simulink model "chapter4_cascaded_nonlinear_closed_pid"  (R2023b)
settings: Solver=ode45  StartTime=0.0  StopTime=100  FixedStep=0.001  MaxStep=1e-3  RelTol=1e-3  EnableMultiTasking=on
values from neighbouring files (symbols this model uses):
  B = 735.75    [rovmodel75kg.mat]
  DL = [3.221 0 0 0 0 0 0 3.291 0 0 0 0 ... (36 elements, 6x6)]    [rovmodel75kg.mat]
  DQ = [105.3 0 0 0 0 0 0 139.6 0 0 0 0 ... (36 elements, 6x6)]    [rovmodel75kg.mat]
  I = [2.51  0  0; 0  3.38  0.01; 0  0.01  1.73]    [rovmodel75kg.mat]
  m = [75  0  0; 0  75  0; 0  0  75]    [rovmodel75kg.mat]
  M = [75 0 0 0 0 0 0 75 0 0 0 0 ... (36 elements, 6x6)]    [rovmodel75kg.mat]
  Ma = [-20.392 0 0 0 0 0 0 -53.435 0 0 0 0 ... (36 elements, 6x6)]    [rovmodel75kg.mat]
  rg = [0 0 0]    [rovmodel75kg.mat]
  W = 735.75    [rovmodel75kg.mat]
  zb = -0.397    [rovmodel75kg.mat]
  zg = 0    [rovmodel75kg.mat]
libraries: simulink_need_slupdate x12
settings Model: Creator=Joshua cheng  LastModifiedBy=yhm
settings SolverCC: AlgebraicLoopSolver=TrustRegion
settings DataIOCC: LimitDataPoints=on  SaveFormat=Array  SignalLoggingSaveFormat=ModelDataLogs  ReturnWorkspaceOutputs=off
settings OptimizationCC: BlockReduction=off  OptimizeBlockIOStorage=off  BufferReuse=off  GlobalBufferReuse=off  ExpressionFolding=off  ExpressionDepthLimit=2147483647  LocalBlockOutputs=off  LifeSpan=inf  OptimizeDataStoreBuffers=off  BusAssignmentInplaceUpdate=off
settings DebuggingCC: SaveWithParameterizedLinksMsg=none  UnderspecifiedInitializationDetection=Classic  MergeDetectMultiDrivingBlocksExec=none  SolverPrmCheckMsg=warning  FcnCallInpInsideContextMsg=warning  UnconnectedInputMsg=warning  UnconnectedOutputMsg=warning  UnconnectedLineMsg=warning  StateNameClashWarn=warning  SFUnexpectedBacktrackingDiag=warning  SFNoUnconditionalDefaultTransitionDiag=warning  SFExecutionAtInitializationDiag=none  ArithmeticOperatorsInVariantConditions=warning
settings HardwareCC: ProdBitPerPointer=32  ProdBitPerSizeT=32  ProdBitPerPtrDiffT=32  ProdLargestAtomicFloat=None  ProdEndianess=BigEndian  ProdWordSize=32  ProdHWDeviceType=Specified  TargetIntDivRoundTo=Zero  TargetEndianess=BigEndian
settings ModelReferenceCC: EnableRefExpFcnMdlSchedulingChecks=on  PropagateSignalLabelsOutOfModel=off
settings SFSimCC: SimUseLocalCustomCode=off  CustomCodeUndefinedFunction=UseInterfaceOnly
settings RTWCC: Description=dSPACE DS1104 Hardware Platform  SystemTargetFile=rti1104.tlc  MakeCommand=make_rti  TemplateMakefile=rti1104.tmf  RTWUseLocalCustomCode=off
settings CodeAppCC: StateflowObjectComments=on
settings STFCustomTargetCC: TargetLangStandard=C89/C90 (ANSI)  MatFileLogging=on  CPPClassGenCompliant=on  GRTInterface=on  SystemTargetFile=rti1104.tlc
settings GRTTargetCC: TargetLangStandard=C89/C90 (ANSI)  ParMdlRefBuildCompliant=off  CompOptLevelCompliant=off  ConcurrentExecutionCompliant=off  CombineOutputUpdateFcns=off  GRTInterface=on  UseToolchainInfoCompliant=off  ExtModeMexFile=noextcomm
settings ConfigComp: CovMetricSettings=dw  CovSaveCumulativeToWorkspaceVar=on  CovSaveSingleToWorkspaceVar=on  CovExternalEMLEnable=off

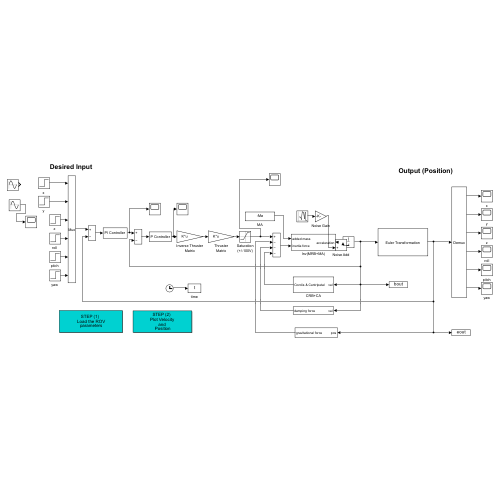
[thumbnail: Simulink's stored preview of the top-level diagram]
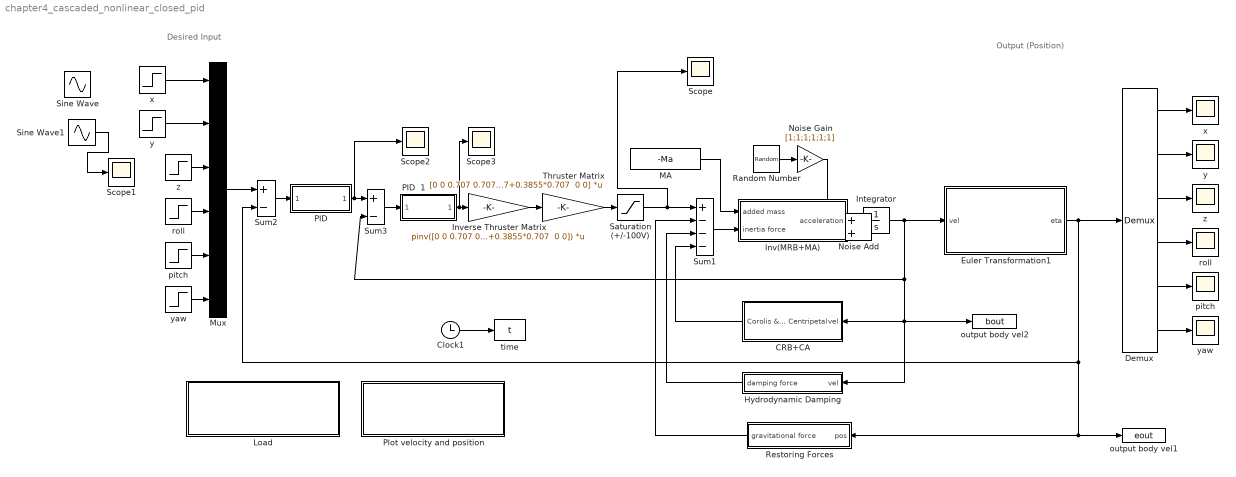
== system chapter4_cascaded_nonlinear_closed_pid ==
  note: Desired Input
  note: Output (Position)
  " Load  " : Subsystem
      settings: OpenFcn=|
      | clc
      | clear all
      | close all
      | load('rovmodel75kg.mat')
      mask Display: disp('STEP (1) \n Load the ROV\n parameters')
  " PID  " : Subsystem  AncestorBlock=|
      | rov_design_analysis/ROV Controller
      | Design
      | Applications/8. PID x 4
      mask Display: disp('PI Controller')
  " PID  1" : Subsystem  AncestorBlock=|
      | rov_design_analysis/ROV Controller
      | Design
      | Applications/8. PID x 4
      mask Display: disp('P Controller')
  CRB+CA : Subsystem
  Clock1 : Clock
  Demux : Demux  Outputs=6
      settings: DisplayOption=none
  Euler Transformation1 : Subsystem  AncestorBlock=rov_design_analysis/Scope Utilities/Euler Transformation
      mask Display: disp('Euler Transformation')
  Hydrodynamic Damping : Subsystem
  Integrator : Integrator  InitialCondition=0.1
  Inv(MRB+MA) : Subsystem
  "Inverse Thruster Matrix " : Gain  Gain=|  Multiplication=Matrix(K*u)  SaturateOnIntegerOverflow=on  OutDataTypeStr=Inherit: Same as input  ParamDataTypeStr=Inherit: Same as input
      | pinv([0 0 0.707 0.707 0 0; 
      |     -0.707 0.707 0.707 -0.707 0 0; 
      |     0.707  0.707  0 0 1 1;
      |     -0.275*0.707+0.4305*0.707 0.275*0.707-0.4305*0.707  0  0  -0.275 0.275;
      |     0.3945*0.707 0.3945*0.707  0.4305*0.707  0.4305*0.707  -0.0355  -0.0355;
      |       -0.3945*0.707  0.3945*0.707  -0.275*0.707-0.3855*0.707  0.275*0.707+0.3855*0.707  0 0])
  MA : Constant  Value=-Ma
  Mux : Mux  Inputs=6
  Noise Add : Sum
  Noise Gain : Gain  Gain=[1;1;1;1;1;1]
  Plot velocity and position : Subsystem  AncestorBlock=|
      | rov_design_analysis/ROV Controller
      | Design
      | Applications/Plot velocity and position
      settings: OpenFcn=|
      | clc
      | 
      | run nonlin_resp6
      mask Display: disp('STEP (2) \n Plot Velocity \n and \n Position')
  Random Number : RandomNumber  Variance=0.001  SampleTime=0.1
  Restoring Forces : Subsystem
  Saturation (+/-100V) : Saturate  UpperLimit=100  LowerLimit=-100
  Scope{,1..3} (4 alike) : Scope
  Sine Wave : Sin  Amplitude=2  Frequency=0.2  Phase=pi/2  SampleTime=0
  Sine Wave1 : Sin  Amplitude=2  Frequency=0.2  SampleTime=0
  Sum1 : Sum  Inputs=+---  InputSameDT=on  SaturateOnIntegerOverflow=on  OutDataTypeStr=Inherit: Same as first input
  Sum2 : Sum  Inputs=+-  InputSameDT=on  SaturateOnIntegerOverflow=on  OutDataTypeStr=Inherit: Same as first input
  Sum3 : Sum  Inputs=+-  InputSameDT=on  SaturateOnIntegerOverflow=on  OutDataTypeStr=Inherit: Same as first input
  "Thruster Matrix " : Gain  Gain=|  Multiplication=Matrix(K*u)  SaturateOnIntegerOverflow=on  OutDataTypeStr=Inherit: Same as input  ParamDataTypeStr=Inherit: Same as input
      | [0 0 0.707 0.707 0 0; 
      |     -0.707 0.707 0.707 -0.707 0 0; 
      |     0.707  0.707  0 0 1 1;
      |     -0.275*0.707+0.4305*0.707 0.275*0.707-0.4305*0.707  0  0  -0.275 0.275;
      |     0.3945*0.707 0.3945*0.707  0.4305*0.707  0.4305*0.707  -0.0355  -0.0355;
      |       -0.3945*0.707  0.3945*0.707  -0.275*0.707-0.3855*0.707  0.275*0.707+0.3855*0.707  0 0]
  output body vel1 : ToWorkspace  VariableName=eout  SampleTime=-1
  output body vel2 : ToWorkspace  VariableName=bout  SampleTime=-1
  pitch : Scope
  "pitch " : Step  Time=0  After=0  SampleTime=0
  roll : Scope
  "roll " : Step  Time=0  After=0  SampleTime=0
  time : ToWorkspace  VariableName=t  SampleTime=-1
  x : Scope
  "x " : Step  Time=0  After=2  SampleTime=0
  y : Scope
  "y " : Step  Time=0  After=2  SampleTime=0
  yaw : Scope
  "yaw " : Step  Time=0  After=0  SampleTime=0
  z : Scope
  "z " : Step  Time=0  After=2  SampleTime=0
  wires:
  Clock1/1 -> time/1
  Euler Transformation1/1("eta ") -> Restoring Forces/1(pos), output body vel1/1, Sum2/2, Demux/1
  MA/1 -> Inv(MRB+MA)/1(added mass)
  CRB+CA/1(Corolis & Centripetal) -> Sum1/4
  Hydrodynamic Damping/1(damping force) -> Sum1/3
  Restoring Forces/1(gravitational force) -> Sum1/2
  Integrator/1 -> CRB+CA/1(vel), Hydrodynamic Damping/1(vel), output body vel2/1, Sum3/2, Euler Transformation1/1(vel)
  Sum1/1 -> Inv(MRB+MA)/2(inertia force)
  "Inverse Thruster Matrix "/1 -> "Thruster Matrix "/1
  "Thruster Matrix "/1 -> Saturation (+/-100V)/1
  "z "/1 -> Mux/3
  "roll "/1 -> Mux/4
  "pitch "/1 -> Mux/5
  "yaw "/1 -> Mux/6
  Demux/6 -> yaw/1
  Demux/3 -> z/1
  Demux/4 -> roll/1
  Demux/5 -> pitch/1
  Demux/2 -> y/1
  Demux/1 -> x/1
  Mux/1 -> Sum2/1
  Sum2/1 -> " PID  "/1(error signal)
  Saturation (+/-100V)/1 -> Scope/1, Sum1/1
  " PID  "/1(control signal) -> Scope2/1, Sum3/1
  " PID  1"/1(control signal) -> Scope3/1, "Inverse Thruster Matrix "/1
  Sum3/1 -> " PID  1"/1(error signal)
  Sine Wave1/1 -> Scope1/1
  "x "/1 -> Mux/1
  "y "/1 -> Mux/2
  Inv(MRB+MA)/1(acceleration) -> Noise Add/1
  Random Number/1 -> Noise Gain/1
  Noise Gain/1 -> Noise Add/2
  Noise Add/1 -> Integrator/1

== system chapter4_cascaded_nonlinear_closed_pid/ Load   ==

== system chapter4_cascaded_nonlinear_closed_pid/ PID   ==
  error signal : Inport
  Demux1 : Demux  Outputs=6
      settings: DisplayOption=none
  Mux2 : Mux  Inputs=6
  PID Controller1 : simulink_need_slupdate/PID Controller  P=2  I=0.5  D=6
  PID Controller2 : simulink_need_slupdate/PID Controller  P=2  I=0.5  D=6
  PID Controller3 : simulink_need_slupdate/PID Controller  P=3  I=0.5  D=6
  PID Controller4 : simulink_need_slupdate/PID Controller  P=3  I=0.5  D=3
  PID Controller5 : simulink_need_slupdate/PID Controller  P=3  I=0.5  D=3
  PID Controller6 : simulink_need_slupdate/PID Controller  P=2  I=0.5  D=6
  control signal : Outport
  wires:
  Mux2/1 -> control signal/1
  error signal/1 -> Demux1/1
  PID Controller2/1 -> Mux2/2
  PID Controller1/1 -> Mux2/1
  Demux1/2 -> PID Controller2/1
  Demux1/1 -> PID Controller1/1
  Demux1/3 -> PID Controller3/1
  PID Controller3/1 -> Mux2/3
  Demux1/6 -> PID Controller6/1
  PID Controller6/1 -> Mux2/6
  Demux1/4 -> PID Controller4/1
  Demux1/5 -> PID Controller5/1
  PID Controller4/1 -> Mux2/4
  PID Controller5/1 -> Mux2/5

== system chapter4_cascaded_nonlinear_closed_pid/ PID  1 ==
  error signal : Inport
  Demux1 : Demux  Outputs=6
      settings: DisplayOption=none
  Mux2 : Mux  Inputs=6
  PID Controller1 : simulink_need_slupdate/PID Controller  P=5  I=0  D=0
  PID Controller2 : simulink_need_slupdate/PID Controller  P=11  I=0  D=0
  PID Controller3 : simulink_need_slupdate/PID Controller  P=12  I=0  D=0
  PID Controller4 : simulink_need_slupdate/PID Controller  P=12  I=0  D=0
  PID Controller5 : simulink_need_slupdate/PID Controller  P=12  I=0  D=0
  PID Controller6 : simulink_need_slupdate/PID Controller  P=11  I=0  D=0
  control signal : Outport
  wires:
  Mux2/1 -> control signal/1
  error signal/1 -> Demux1/1
  PID Controller2/1 -> Mux2/2
  PID Controller1/1 -> Mux2/1
  Demux1/2 -> PID Controller2/1
  Demux1/1 -> PID Controller1/1
  Demux1/3 -> PID Controller3/1
  PID Controller3/1 -> Mux2/3
  Demux1/6 -> PID Controller6/1
  PID Controller6/1 -> Mux2/6
  Demux1/4 -> PID Controller4/1
  Demux1/5 -> PID Controller5/1
  PID Controller4/1 -> Mux2/4
  PID Controller5/1 -> Mux2/5

== system chapter4_cascaded_nonlinear_closed_pid/CRB+CA ==
  vel : Inport
  Add : Sum
  Centripetal & Coriolis : Subsystem  AncestorBlock=rov_design_analysis/ROV Models/1. Six DOF RRC ROV II/Centripetal & Coriolis
      mask Display: disp('CRB')
  Centripetal & Coriolis1 : Subsystem  AncestorBlock=rov_design_analysis/ROV Models/1. Six DOF RRC ROV II/Centripetal & Coriolis
      mask Display: disp('CA')
  Corolis & Centripetal : Outport
  wires:
  vel/1 -> Centripetal & Coriolis/1(vel), Centripetal & Coriolis1/1(vel)
  Add/1 -> Corolis & Centripetal/1
  Centripetal & Coriolis/1(force) -> Add/1
  Centripetal & Coriolis1/1(force) -> Add/2

== system chapter4_cascaded_nonlinear_closed_pid/Euler Transformation1 ==
  vel : Inport
  1/s : Subsystem
  Demux : Demux  Outputs=2
      settings: DisplayOption=none
  Demux1 : Demux  Outputs=2
      settings: DisplayOption=none
  Mux1 : Mux  Inputs=2
  Saturation : Saturate  UpperLimit=360  LowerLimit=-360
  Terminator : Terminator
  Transformation matrix R : Subsystem
      mask Display: disp('Transformation R')
  Transformation matrix T : Subsystem
      mask Display: disp('Transformation T')
  "eta " : Outport  InitialOutput=0
  wires:
  Mux1/1 -> 1/s/1(In1)
  Demux/2 -> Transformation matrix R/1(angular body velocity)
  Demux/1 -> Transformation matrix T/1(translational body velocity)
  vel/1 -> Demux/1
  Demux1/2 -> Transformation matrix T/2(angular position), Transformation matrix R/2(angular position)
  Transformation matrix R/1(angular earth velocity) -> Mux1/2
  Transformation matrix T/1(translational earth velocity) -> Mux1/1
  Demux1/1 -> Terminator/1
  1/s/1(Out1) -> Saturation/1
  Saturation/1 -> Demux1/1, "eta "/1

== system chapter4_cascaded_nonlinear_closed_pid/Hydrodynamic Damping ==
  vel : Inport
  Abs : Abs  SaturateOnIntegerOverflow=off
  Add : Sum
  Constant : Constant  Value=0
  D linear : Gain  Gain=diag(DL)  SaturateOnIntegerOverflow=on  OutDataTypeStr=Inherit: Same as input  ParamDataTypeStr=Inherit: Same as input
  D quadratic : Gain  Gain=diag(DQ)  SaturateOnIntegerOverflow=on  OutDataTypeStr=Inherit: Same as input  ParamDataTypeStr=Inherit: Same as input
  Manual Switch : ManualSwitch  CurrentSetting=0
  Manual Switch1 : ManualSwitch  CurrentSetting=0
  Product : Product  RndMeth=Zero
  damping force : Outport  InitialOutput=0
  wires:
  vel/1 -> D linear/1, Abs/1, Product/2
  D linear/1 -> Manual Switch/1
  Add/1 -> damping force/1
  Abs/1 -> D quadratic/1
  D quadratic/1 -> Product/1
  Manual Switch/1 -> Add/1
  Product/1 -> Manual Switch/2, Manual Switch1/2
  Manual Switch1/1 -> Add/2
  Constant/1 -> Manual Switch1/1

== system chapter4_cascaded_nonlinear_closed_pid/Inv(MRB+MA) ==
  added mass : Inport
  inertia force : Inport  Port=2
  Display : Display
      settings: Decimation=2
  Display2 : Display
      settings: Decimation=2
  Divide : Product  Inputs=/  Multiplication=Matrix(*)
  MRB - open : Constant  Value=M
  Product : Product  Multiplication=Matrix(*)  RndMeth=Zero
  Sum1 : Sum  InputSameDT=on  SaturateOnIntegerOverflow=on  OutDataTypeStr=Inherit: Same as first input
  acceleration : Outport
  wires:
  Divide/1 -> Display/1, Product/1
  Product/1 -> acceleration/1, Display2/1
  inertia force/1 -> Product/2
  added mass/1 -> Sum1/2
  Sum1/1 -> Divide/1
  MRB - open/1 -> Sum1/1

== system chapter4_cascaded_nonlinear_closed_pid/Plot velocity and position ==

== system chapter4_cascaded_nonlinear_closed_pid/Restoring Forces ==
  pos : Inport
  (zg.W - zb.B)cY.sX : Fcn  Expr=((zg * W - zb * B) * cos(u[2])) * sin(u[1])
  (zg.W - zb.B)sY : Fcn  Expr=(zg*W - zb*B)*sin(u[2])
  -(xg.W-xb.B)cY.sX : Fcn  Expr=0
  -cY.cX : Fcn  Expr=0
  -cY.sX : Fcn  Expr=0
  Demux : Demux  Outputs=2
      settings: DisplayOption=none
  Mux1 : Mux  Inputs=6
  Terminator : Terminator
  sY : Fcn  Expr=0
  gravitational force : Outport  InitialOutput=0
  wires:
  Mux1/1 -> gravitational force/1
  Demux/2 -> (zg.W - zb.B)cY.sX/1, (zg.W - zb.B)sY/1, -(xg.W-xb.B)cY.sX/1, sY/1, -cY.sX/1, -cY.cX/1  "pos_2"
  Demux/1 -> Terminator/1  "pos_1"
  pos/1 -> Demux/1
  sY/1 -> Mux1/1
  -cY.sX/1 -> Mux1/2
  -cY.cX/1 -> Mux1/3
  (zg.W - zb.B)cY.sX/1 -> Mux1/4
  (zg.W - zb.B)sY/1 -> Mux1/5
  -(xg.W-xb.B)cY.sX/1 -> Mux1/6

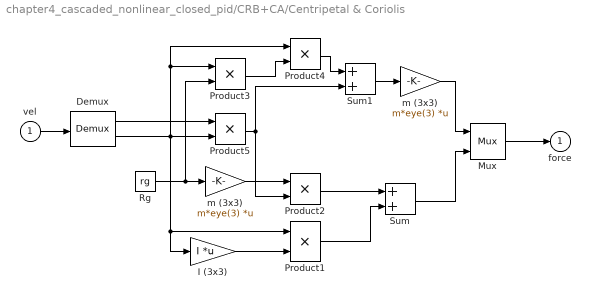
== system chapter4_cascaded_nonlinear_closed_pid/CRB+CA/Centripetal & Coriolis ==
  vel : Inport
  Demux : Demux  Outputs=2
      settings: DisplayOption=none
  "I (3x3) " : Gain  Gain=I  Multiplication=Matrix(K*u)  SaturateOnIntegerOverflow=on  OutDataTypeStr=Inherit: Same as input  ParamDataTypeStr=Inherit: Same as input
  Mux : Mux  Inputs=2
  Product{1..5} (5 alike) : Product  InputSameDT=on  RndMeth=Zero  SaturateOnIntegerOverflow=on  OutDataTypeStr=Inherit: Same as first input
  Rg : Constant  Value=rg
  Sum : Sum  InputSameDT=on  SaturateOnIntegerOverflow=on  OutDataTypeStr=Inherit: Same as first input
  Sum1 : Sum  InputSameDT=on  SaturateOnIntegerOverflow=on  OutDataTypeStr=Inherit: Same as first input
  m (3x3) : Gain  Gain=m*eye(3)  Multiplication=Matrix(K*u)  SaturateOnIntegerOverflow=on  OutDataTypeStr=Inherit: Same as input  ParamDataTypeStr=Inherit: Same as input
  "m (3x3) " : Gain  Gain=m*eye(3)  Multiplication=Matrix(K*u)  SaturateOnIntegerOverflow=on  OutDataTypeStr=Inherit: Same as input  ParamDataTypeStr=Inherit: Same as input
  force : Outport  InitialOutput=0
  wires:
  Product1/1 -> Sum/2
  "m (3x3) "/1 -> Product2/1
  Product2/1 -> Sum/1
  Product3/1 -> Product4/2
  Product4/1 -> Sum1/1
  Product5/1 -> Product2/2, Sum1/2
  Sum1/1 -> m (3x3)/1
  vel/1 -> Demux/1
  m (3x3)/1 -> Mux/1
  Sum/1 -> Mux/2
  Mux/1 -> force/1
  Demux/1 -> Product5/1
  Demux/2 -> Product5/2, Product3/1, Product4/1, Product1/1, "I (3x3) "/1
  Rg/1 -> "m (3x3) "/1, Product3/2
  "I (3x3) "/1 -> Product1/2

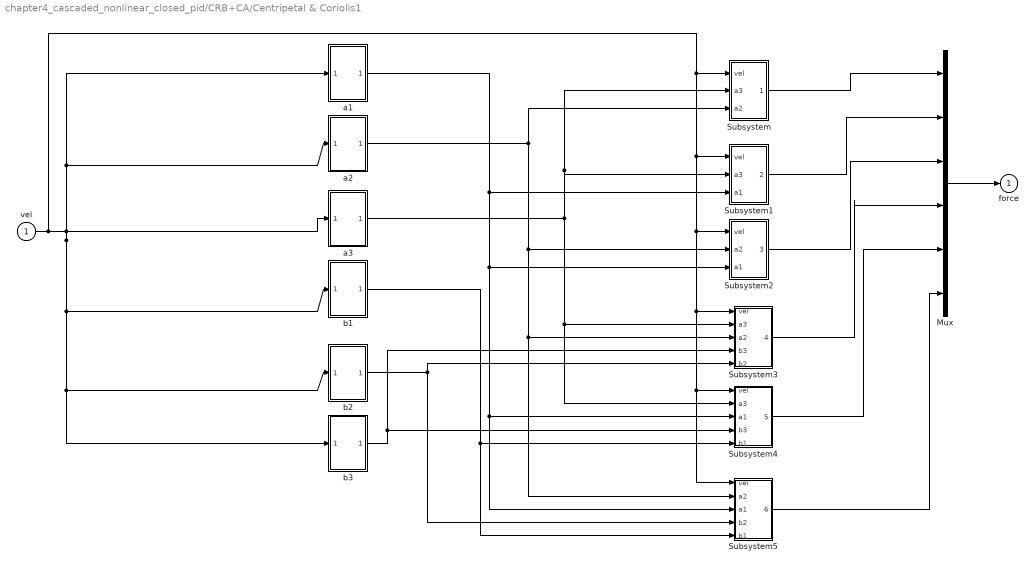
== system chapter4_cascaded_nonlinear_closed_pid/CRB+CA/Centripetal & Coriolis1 ==
  vel : Inport
  Mux : Mux  Inputs=6
  Subsystem : Subsystem
  Subsystem1 : Subsystem
  Subsystem2 : Subsystem
  Subsystem3 : Subsystem
  Subsystem4 : Subsystem
  Subsystem5 : Subsystem
  a1 : Subsystem
      mask Display: disp('Row 1')
  a2 : Subsystem
      mask Display: disp('Row 2')
  a3 : Subsystem
      mask Display: disp('Row 1')
  b1 : Subsystem
      mask Display: disp('Row 2')
  b2 : Subsystem
      mask Display: disp('Row 1')
  b3 : Subsystem
      mask Display: disp('Row 2')
  force : Outport  InitialOutput=0
  wires:
  vel/1 -> a1/1(In1), a2/1(In1), a3/1(In1), b1/1(In1), b2/1(In1), b3/1(In1), Subsystem/1(vel), Subsystem1/1(vel), Subsystem2/1(vel), Subsystem3/1(vel), Subsystem4/1(vel), Subsystem5/1(vel)
  Mux/1 -> force/1
  Subsystem/1(1) -> Mux/1
  Subsystem1/1(2) -> Mux/2
  Subsystem2/1(3) -> Mux/3
  Subsystem3/1(4) -> Mux/4
  Subsystem4/1(5) -> Mux/5
  Subsystem5/1(6) -> Mux/6
  a3/1(Out1) -> Subsystem/2(a3), Subsystem1/2(a3), Subsystem3/2(a3), Subsystem4/2(a3)
  a2/1(Out1) -> Subsystem/3(a2), Subsystem2/2(a2), Subsystem3/3(a2), Subsystem5/2("a2 ")
  b1/1(Out1) -> Subsystem4/5(b1), Subsystem5/5("b1 ")
  a1/1(Out1) -> Subsystem1/3(a1), Subsystem2/3(a1), Subsystem4/3(a1), Subsystem5/3("a1 ")
  b2/1(Out1) -> Subsystem5/4("b2 "), Subsystem3/5(b2)
  b3/1(Out1) -> Subsystem4/4(b3), Subsystem3/4(b3)

== system chapter4_cascaded_nonlinear_closed_pid/Euler Transformation1/1//s ==
  In1 : Inport
  Demux2 : Demux  Outputs=6
      settings: DisplayOption=none
  Integrator{,1..2,4..6} (6 alike) : Integrator
  Mux2 : Mux  Inputs=6
  Out1 : Outport
  wires:
  Demux2/1 -> Integrator/1
  Demux2/2 -> Integrator1/1
  Demux2/3 -> Integrator2/1
  Demux2/4 -> Integrator4/1
  Demux2/5 -> Integrator5/1
  Integrator/1 -> Mux2/1
  Integrator1/1 -> Mux2/2
  Integrator2/1 -> Mux2/3
  Integrator4/1 -> Mux2/4
  In1/1 -> Demux2/1
  Mux2/1 -> Out1/1
  Integrator5/1 -> Mux2/5
  Demux2/6 -> Integrator6/1
  Integrator6/1 -> Mux2/6

== system chapter4_cascaded_nonlinear_closed_pid/Euler Transformation1/Transformation matrix R ==
  angular body velocity : Inport
  angular position : Inport  Port=2
  Mux : Mux  Inputs=3
  Row1 of T : Subsystem
      mask Display: disp('Row 1')
  Row2 of T : Subsystem
      mask Display: disp('Row 2')
  Row3 of T : Subsystem
      mask Display: disp('Row 3')
  angular earth velocity : Outport
  wires:
  angular position/1 -> Row3 of T/2(angular position), Row1 of T/2(angular position), Row2 of T/2(angular position)
  Mux/1 -> angular earth velocity/1
  Row3 of T/1(angular earth velocity (row 3)) -> Mux/3
  angular body velocity/1 -> Row1 of T/1(angular body velocity), Row3 of T/1("angular body velocity "), Row2 of T/1("angular body velocity ")
  Row2 of T/1(angular earth velocity (row 2)) -> Mux/2
  Row1 of T/1(angular earth velocity (row 1)) -> Mux/1

== system chapter4_cascaded_nonlinear_closed_pid/Euler Transformation1/Transformation matrix T ==
  translational body velocity : Inport
  angular position : Inport  Port=2
  Mux : Mux  Inputs=3
  Row1 of R : Subsystem
      mask Display: disp('Row 1')
  Row2 of R : Subsystem
      mask Display: disp('Row 2')
  Row3 of R : Subsystem
      mask Display: disp('Row 3')
  translational earth velocity : Outport  InitialOutput=0
  wires:
  Mux/1 -> translational earth velocity/1
  Row3 of R/1(translational earth velocity (row 3)) -> Mux/3
  Row2 of R/1(translational earth velocity (row 2)) -> Mux/2
  angular position/1 -> Row3 of R/2(angular position), Row1 of R/2(angular position), Row2 of R/2(angular position)
  translational body velocity/1 -> Row1 of R/1(translational body velocity), Row2 of R/1(translational body velocity), Row3 of R/1(translational body velocity)
  Row1 of R/1(translational earth velocity (row 1)) -> Mux/1

== system chapter4_cascaded_nonlinear_closed_pid/CRB+CA/Centripetal & Coriolis1/Subsystem ==
  vel : Inport
  a3 : Inport  Port=2
  a2 : Inport  Port=3
  Add : Sum
  Demux : Demux  Outputs=6
  Gain : Gain  Gain=-1
  Product : Product  RndMeth=Zero
  Product1 : Product  RndMeth=Zero
  1 : Outport
  wires:
  Demux/6 -> Product1/2
  Product1/1 -> Add/2
  Product/1 -> Add/1
  Demux/5 -> Gain/1
  Gain/1 -> Product/1
  vel/1 -> Demux/1
  a3/1 -> Product/2
  Add/1 -> 1/1
  a2/1 -> Product1/1

== system chapter4_cascaded_nonlinear_closed_pid/CRB+CA/Centripetal & Coriolis1/Subsystem1 ==
  vel : Inport
  a3 : Inport  Port=2
  a1 : Inport  Port=3
  Add : Sum
  Demux : Demux  Outputs=6
  Gain : Gain
  Gain1 : Gain  Gain=-1
  Product : Product  RndMeth=Zero
  Product1 : Product  RndMeth=Zero
  2 : Outport
  wires:
  Demux/6 -> Gain1/1
  Product1/1 -> Add/2
  Product/1 -> Add/1
  Gain/1 -> Product/1
  vel/1 -> Demux/1
  a3/1 -> Product/2
  Add/1 -> 2/1
  a1/1 -> Product1/1
  Gain1/1 -> Product1/2
  Demux/4 -> Gain/1

== system chapter4_cascaded_nonlinear_closed_pid/CRB+CA/Centripetal & Coriolis1/Subsystem2 ==
  vel : Inport
  a2 : Inport  Port=2
  a1 : Inport  Port=3
  Add : Sum
  Demux : Demux  Outputs=6
  Gain : Gain  Gain=-1
  Gain1 : Gain
  Product : Product  RndMeth=Zero
  Product1 : Product  RndMeth=Zero
  3 : Outport
  wires:
  Product1/1 -> Add/2
  Product/1 -> Add/1
  Gain/1 -> Product/1
  vel/1 -> Demux/1
  a2/1 -> Product/2
  Add/1 -> 3/1
  a1/1 -> Product1/1
  Gain1/1 -> Product1/2
  Demux/4 -> Gain/1
  Demux/5 -> Gain1/1

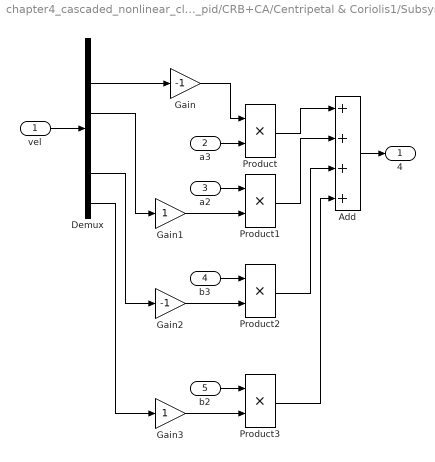
== system chapter4_cascaded_nonlinear_closed_pid/CRB+CA/Centripetal & Coriolis1/Subsystem3 ==
  vel : Inport
  a3 : Inport  Port=2
  a2 : Inport  Port=3
  b3 : Inport  Port=4
  b2 : Inport  Port=5
  Add : Sum  Inputs=++++
  Demux : Demux  Outputs=6
  Gain : Gain  Gain=-1
  Gain1 : Gain
  Gain2 : Gain  Gain=-1
  Gain3 : Gain
  Product{,1..3} (4 alike) : Product  RndMeth=Zero
  4 : Outport
  wires:
  Product1/1 -> Add/2
  Product/1 -> Add/1
  Gain/1 -> Product/1
  vel/1 -> Demux/1
  a3/1 -> Product/2
  Add/1 -> 4/1
  a2/1 -> Product1/1
  Gain1/1 -> Product1/2
  Demux/2 -> Gain/1
  Demux/3 -> Gain1/1
  b3/1 -> Product2/1
  Gain2/1 -> Product2/2
  b2/1 -> Product3/1
  Gain3/1 -> Product3/2
  Demux/5 -> Gain2/1
  Demux/6 -> Gain3/1
  Product2/1 -> Add/3
  Product3/1 -> Add/4

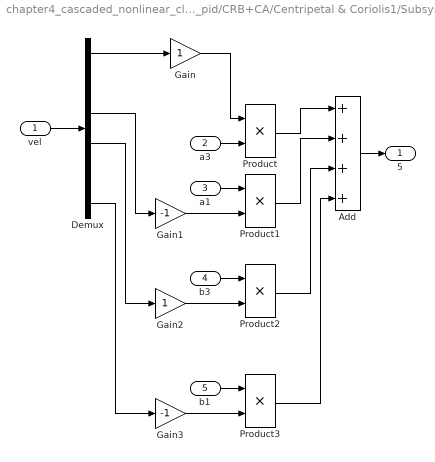
== system chapter4_cascaded_nonlinear_closed_pid/CRB+CA/Centripetal & Coriolis1/Subsystem4 ==
  vel : Inport
  a3 : Inport  Port=2
  a1 : Inport  Port=3
  b3 : Inport  Port=4
  b1 : Inport  Port=5
  Add : Sum  Inputs=++++
  Demux : Demux  Outputs=6
  Gain : Gain
  Gain1 : Gain  Gain=-1
  Gain2 : Gain
  Gain3 : Gain  Gain=-1
  Product{,1..3} (4 alike) : Product  RndMeth=Zero
  5 : Outport
  wires:
  Product1/1 -> Add/2
  Product/1 -> Add/1
  Gain/1 -> Product/1
  vel/1 -> Demux/1
  a3/1 -> Product/2
  Add/1 -> 5/1
  a1/1 -> Product1/1
  Gain1/1 -> Product1/2
  Demux/3 -> Gain1/1
  b3/1 -> Product2/1
  Gain2/1 -> Product2/2
  b1/1 -> Product3/1
  Gain3/1 -> Product3/2
  Demux/6 -> Gain3/1
  Product2/1 -> Add/3
  Product3/1 -> Add/4
  Demux/1 -> Gain/1
  Demux/4 -> Gain2/1

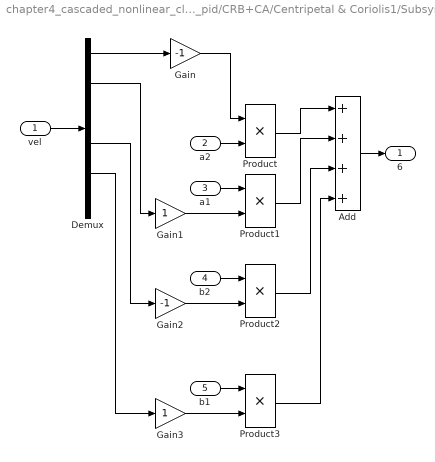
== system chapter4_cascaded_nonlinear_closed_pid/CRB+CA/Centripetal & Coriolis1/Subsystem5 ==
  vel : Inport
  "a2 " : Inport  Port=2
  "a1 " : Inport  Port=3
  "b2 " : Inport  Port=4
  "b1 " : Inport  Port=5
  Add : Sum  Inputs=++++
  Demux : Demux  Outputs=6
  Gain : Gain  Gain=-1
  Gain1 : Gain
  Gain2 : Gain  Gain=-1
  Gain3 : Gain
  Product{,1..3} (4 alike) : Product  RndMeth=Zero
  6 : Outport
  wires:
  Product1/1 -> Add/2
  Product/1 -> Add/1
  Gain/1 -> Product/1
  vel/1 -> Demux/1
  "a2 "/1 -> Product/2
  Add/1 -> 6/1
  "a1 "/1 -> Product1/1
  Gain1/1 -> Product1/2
  "b2 "/1 -> Product2/1
  Gain2/1 -> Product2/2
  "b1 "/1 -> Product3/1
  Gain3/1 -> Product3/2
  Product2/1 -> Add/3
  Product3/1 -> Add/4
  Demux/1 -> Gain/1
  Demux/2 -> Gain1/1
  Demux/4 -> Gain2/1
  Demux/5 -> Gain3/1

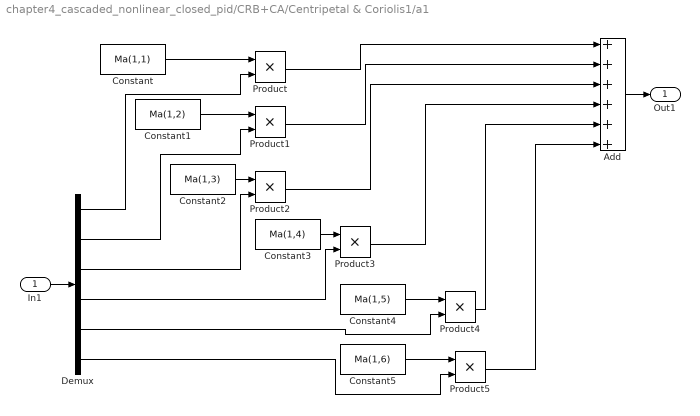
== system chapter4_cascaded_nonlinear_closed_pid/CRB+CA/Centripetal & Coriolis1/a1 ==
  In1 : Inport
  Add : Sum  Inputs=++++++
  Constant : Constant  Value=Ma(1,1)
  Constant1 : Constant  Value=Ma(1,2)
  Constant2 : Constant  Value=Ma(1,3)
  Constant3 : Constant  Value=Ma(1,4)
  Constant4 : Constant  Value=Ma(1,5)
  Constant5 : Constant  Value=Ma(1,6)
  Demux : Demux  Outputs=6
  Product{,1..5} (6 alike) : Product  RndMeth=Zero
  Out1 : Outport
  wires:
  Demux/1 -> Product/2
  Demux/2 -> Product1/2
  Demux/3 -> Product2/2
  Demux/4 -> Product3/2
  Demux/5 -> Product4/2
  Demux/6 -> Product5/2
  Product5/1 -> Add/6
  Constant5/1 -> Product5/1
  Product4/1 -> Add/5
  Constant4/1 -> Product4/1
  Product3/1 -> Add/4
  Constant3/1 -> Product3/1
  Product2/1 -> Add/3
  Constant2/1 -> Product2/1
  Product1/1 -> Add/2
  Constant1/1 -> Product1/1
  Product/1 -> Add/1
  Constant/1 -> Product/1
  Add/1 -> Out1/1
  In1/1 -> Demux/1

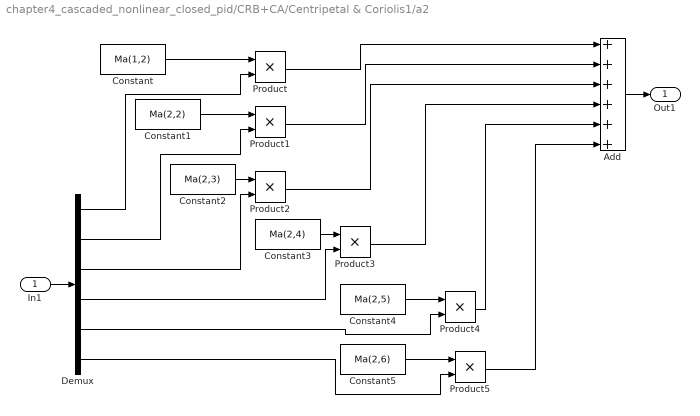
== system chapter4_cascaded_nonlinear_closed_pid/CRB+CA/Centripetal & Coriolis1/a2 ==
  In1 : Inport
  Add : Sum  Inputs=++++++
  Constant : Constant  Value=Ma(1,2)
  Constant1 : Constant  Value=Ma(2,2)
  Constant2 : Constant  Value=Ma(2,3)
  Constant3 : Constant  Value=Ma(2,4)
  Constant4 : Constant  Value=Ma(2,5)
  Constant5 : Constant  Value=Ma(2,6)
  Demux : Demux  Outputs=6
  Product{,1..5} (6 alike) : Product  RndMeth=Zero
  Out1 : Outport
  wires:
  Demux/1 -> Product/2
  Demux/2 -> Product1/2
  Demux/3 -> Product2/2
  Demux/4 -> Product3/2
  Demux/5 -> Product4/2
  Demux/6 -> Product5/2
  Product5/1 -> Add/6
  Constant5/1 -> Product5/1
  Product4/1 -> Add/5
  Constant4/1 -> Product4/1
  Product3/1 -> Add/4
  Constant3/1 -> Product3/1
  Product2/1 -> Add/3
  Constant2/1 -> Product2/1
  Product1/1 -> Add/2
  Constant1/1 -> Product1/1
  Product/1 -> Add/1
  Constant/1 -> Product/1
  Add/1 -> Out1/1
  In1/1 -> Demux/1

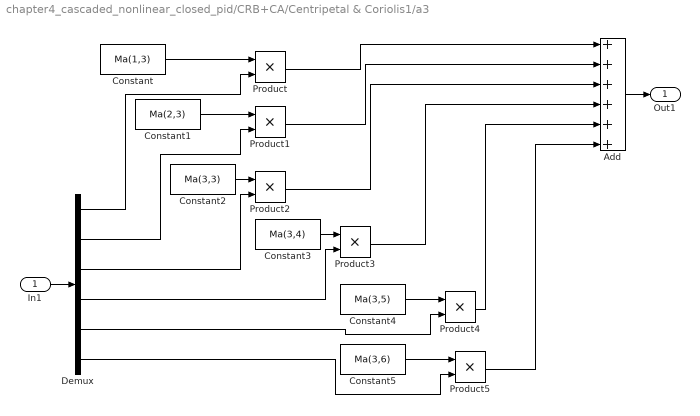
== system chapter4_cascaded_nonlinear_closed_pid/CRB+CA/Centripetal & Coriolis1/a3 ==
  In1 : Inport
  Add : Sum  Inputs=++++++
  Constant : Constant  Value=Ma(1,3)
  Constant1 : Constant  Value=Ma(2,3)
  Constant2 : Constant  Value=Ma(3,3)
  Constant3 : Constant  Value=Ma(3,4)
  Constant4 : Constant  Value=Ma(3,5)
  Constant5 : Constant  Value=Ma(3,6)
  Demux : Demux  Outputs=6
  Product{,1..5} (6 alike) : Product  RndMeth=Zero
  Out1 : Outport
  wires:
  Demux/1 -> Product/2
  Demux/2 -> Product1/2
  Demux/3 -> Product2/2
  Demux/4 -> Product3/2
  Demux/5 -> Product4/2
  Demux/6 -> Product5/2
  Product5/1 -> Add/6
  Constant5/1 -> Product5/1
  Product4/1 -> Add/5
  Constant4/1 -> Product4/1
  Product3/1 -> Add/4
  Constant3/1 -> Product3/1
  Product2/1 -> Add/3
  Constant2/1 -> Product2/1
  Product1/1 -> Add/2
  Constant1/1 -> Product1/1
  Product/1 -> Add/1
  Constant/1 -> Product/1
  Add/1 -> Out1/1
  In1/1 -> Demux/1

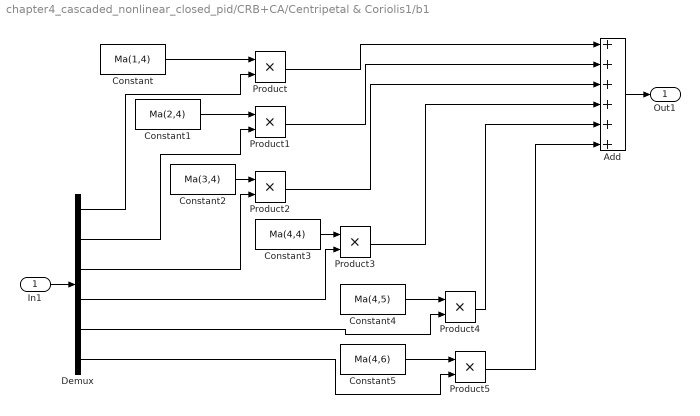
== system chapter4_cascaded_nonlinear_closed_pid/CRB+CA/Centripetal & Coriolis1/b1 ==
  In1 : Inport
  Add : Sum  Inputs=++++++
  Constant : Constant  Value=Ma(1,4)
  Constant1 : Constant  Value=Ma(2,4)
  Constant2 : Constant  Value=Ma(3,4)
  Constant3 : Constant  Value=Ma(4,4)
  Constant4 : Constant  Value=Ma(4,5)
  Constant5 : Constant  Value=Ma(4,6)
  Demux : Demux  Outputs=6
  Product{,1..5} (6 alike) : Product  RndMeth=Zero
  Out1 : Outport
  wires:
  Demux/1 -> Product/2
  Demux/2 -> Product1/2
  Demux/3 -> Product2/2
  Demux/4 -> Product3/2
  Demux/5 -> Product4/2
  Demux/6 -> Product5/2
  Product5/1 -> Add/6
  Constant5/1 -> Product5/1
  Product4/1 -> Add/5
  Constant4/1 -> Product4/1
  Product3/1 -> Add/4
  Constant3/1 -> Product3/1
  Product2/1 -> Add/3
  Constant2/1 -> Product2/1
  Product1/1 -> Add/2
  Constant1/1 -> Product1/1
  Product/1 -> Add/1
  Constant/1 -> Product/1
  Add/1 -> Out1/1
  In1/1 -> Demux/1

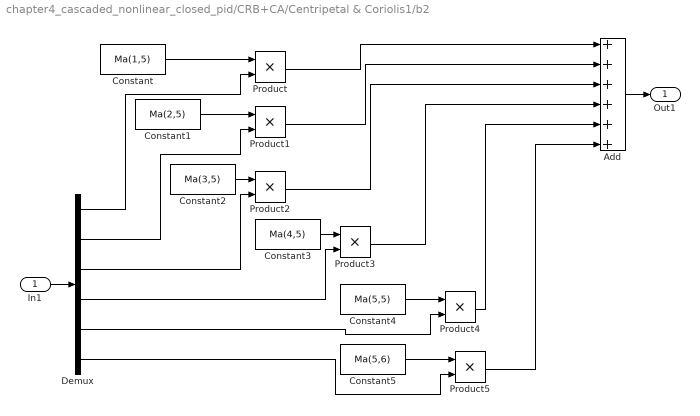
== system chapter4_cascaded_nonlinear_closed_pid/CRB+CA/Centripetal & Coriolis1/b2 ==
  In1 : Inport
  Add : Sum  Inputs=++++++
  Constant : Constant  Value=Ma(1,5)
  Constant1 : Constant  Value=Ma(2,5)
  Constant2 : Constant  Value=Ma(3,5)
  Constant3 : Constant  Value=Ma(4,5)
  Constant4 : Constant  Value=Ma(5,5)
  Constant5 : Constant  Value=Ma(5,6)
  Demux : Demux  Outputs=6
  Product{,1..5} (6 alike) : Product  RndMeth=Zero
  Out1 : Outport
  wires:
  Demux/1 -> Product/2
  Demux/2 -> Product1/2
  Demux/3 -> Product2/2
  Demux/4 -> Product3/2
  Demux/5 -> Product4/2
  Demux/6 -> Product5/2
  Product5/1 -> Add/6
  Constant5/1 -> Product5/1
  Product4/1 -> Add/5
  Constant4/1 -> Product4/1
  Product3/1 -> Add/4
  Constant3/1 -> Product3/1
  Product2/1 -> Add/3
  Constant2/1 -> Product2/1
  Product1/1 -> Add/2
  Constant1/1 -> Product1/1
  Product/1 -> Add/1
  Constant/1 -> Product/1
  Add/1 -> Out1/1
  In1/1 -> Demux/1

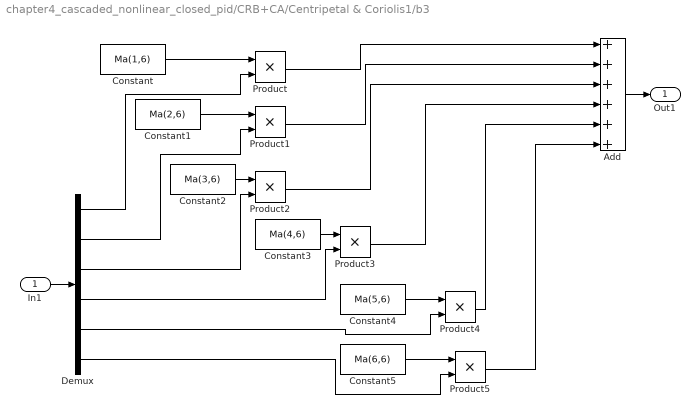
== system chapter4_cascaded_nonlinear_closed_pid/CRB+CA/Centripetal & Coriolis1/b3 ==
  In1 : Inport
  Add : Sum  Inputs=++++++
  Constant : Constant  Value=Ma(1,6)
  Constant1 : Constant  Value=Ma(2,6)
  Constant2 : Constant  Value=Ma(3,6)
  Constant3 : Constant  Value=Ma(4,6)
  Constant4 : Constant  Value=Ma(5,6)
  Constant5 : Constant  Value=Ma(6,6)
  Demux : Demux  Outputs=6
  Product{,1..5} (6 alike) : Product  RndMeth=Zero
  Out1 : Outport
  wires:
  Demux/1 -> Product/2
  Demux/2 -> Product1/2
  Demux/3 -> Product2/2
  Demux/4 -> Product3/2
  Demux/5 -> Product4/2
  Demux/6 -> Product5/2
  Product5/1 -> Add/6
  Constant5/1 -> Product5/1
  Product4/1 -> Add/5
  Constant4/1 -> Product4/1
  Product3/1 -> Add/4
  Constant3/1 -> Product3/1
  Product2/1 -> Add/3
  Constant2/1 -> Product2/1
  Product1/1 -> Add/2
  Constant1/1 -> Product1/1
  Product/1 -> Add/1
  Constant/1 -> Product/1
  Add/1 -> Out1/1
  In1/1 -> Demux/1

== system chapter4_cascaded_nonlinear_closed_pid/Euler Transformation1/Transformation matrix R/Row1 of T ==
  angular body velocity : Inport
  angular position : Inport  Port=2
  1 : Fcn  Expr=1
  Dot Product : DotProduct  OutDataTypeStr=Inherit: Inherit via internal rule
  Mux1 : Mux  Inputs=3
  cX.tY : Fcn  Expr=cos(u[1])*tan(u[2])
  sX.tY : Fcn  Expr=sin(u[1])*tan(u[2])
  angular earth velocity (row 1) : Outport
  wires:
  Mux1/1 -> Dot Product/1
  cX.tY/1 -> Mux1/3
  sX.tY/1 -> Mux1/2
  1/1 -> Mux1/1
  angular position/1 -> cX.tY/1, sX.tY/1, 1/1
  angular body velocity/1 -> Dot Product/2
  Dot Product/1 -> angular earth velocity (row 1)/1

== system chapter4_cascaded_nonlinear_closed_pid/Euler Transformation1/Transformation matrix R/Row2 of T ==
  "angular body velocity " : Inport
  angular position : Inport  Port=2
  -sX : Fcn  Expr=-sin(u[1])
  0 : Fcn  Expr=0
  Dot Product : DotProduct  OutDataTypeStr=Inherit: Inherit via internal rule
  Dot Product1 : Subsystem
  Mux1 : Mux  Inputs=3
  cX : Fcn  Expr=cos(u[1])
  angular earth velocity (row 2) : Outport
  wires:
  Mux1/1 -> Dot Product/1
  -sX/1 -> Mux1/3
  cX/1 -> Mux1/2
  0/1 -> Mux1/1
  angular position/1 -> -sX/1, cX/1, 0/1
  "angular body velocity "/1 -> Dot Product/2
  Dot Product/1 -> angular earth velocity (row 2)/1

== system chapter4_cascaded_nonlinear_closed_pid/Euler Transformation1/Transformation matrix R/Row3 of T ==
  "angular body velocity " : Inport
  angular position : Inport  Port=2
  1 : Fcn  Expr=0
  Dot Product : DotProduct  OutDataTypeStr=Inherit: Inherit via internal rule
  Mux1 : Mux  Inputs=3
  cX/cY : Fcn  Expr=cos(u[1])/cos(u[2])
  sX/cY : Fcn  Expr=sin(u[1])/cos(u[2])
  angular earth velocity (row 3) : Outport
  wires:
  Mux1/1 -> Dot Product/1
  cX/cY/1 -> Mux1/3
  sX/cY/1 -> Mux1/2
  1/1 -> Mux1/1
  angular position/1 -> cX/cY/1, sX/cY/1, 1/1
  "angular body velocity "/1 -> Dot Product/2
  Dot Product/1 -> angular earth velocity (row 3)/1

== system chapter4_cascaded_nonlinear_closed_pid/Euler Transformation1/Transformation matrix T/Row1 of R ==
  translational body velocity : Inport
  angular position : Inport  Port=2
  -sZ.cX+cZ.sY.sX : Fcn  Expr=-sin(u[3])*cos(u[1]) + cos(u[3])*sin(u[2])*sin(u[1])
  Dot Product : DotProduct  OutDataTypeStr=Inherit: Inherit via internal rule
  Mux : Mux  Inputs=3
  cY.cZ : Fcn  Expr=cos(u[3]) * cos(u[2])
  sZ.sX+cZ.cX.sY : Fcn  Expr=sin(u[3])*sin(u[1]) + cos(u[3])*cos(u[1])*sin(u[2])
  translational earth velocity (row 1) : Outport
  wires:
  translational body velocity/1 -> Dot Product/2
  Mux/1 -> Dot Product/1
  sZ.sX+cZ.cX.sY/1 -> Mux/3
  -sZ.cX+cZ.sY.sX/1 -> Mux/2
  cY.cZ/1 -> Mux/1
  angular position/1 -> sZ.sX+cZ.cX.sY/1, -sZ.cX+cZ.sY.sX/1, cY.cZ/1
  Dot Product/1 -> translational earth velocity (row 1)/1

== system chapter4_cascaded_nonlinear_closed_pid/Euler Transformation1/Transformation matrix T/Row2 of R ==
  translational body velocity : Inport
  angular position : Inport  Port=2
  -cZ.sX+sY.sZ.cX : Fcn  Expr=-cos(u[3])*sin(u[1]) + sin(u[2])*sin(u[3])*cos(u[1])
  Dot Product : DotProduct  OutDataTypeStr=Inherit: Inherit via internal rule
  Mux1 : Mux  Inputs=3
  cY.sZ : Fcn  Expr=sin(u[3]) * cos(u[2])
  cZ.cX+sX.sY.sZ : Fcn  Expr=cos(u[3])*cos(u[1]) + sin(u[1])*sin(u[2])*sin(u[3])
  translational earth velocity (row 2) : Outport
  wires:
  -cZ.sX+sY.sZ.cX/1 -> Mux1/3
  cZ.cX+sX.sY.sZ/1 -> Mux1/2
  cY.sZ/1 -> Mux1/1
  angular position/1 -> -cZ.sX+sY.sZ.cX/1, cZ.cX+sX.sY.sZ/1, cY.sZ/1
  Mux1/1 -> Dot Product/1
  translational body velocity/1 -> Dot Product/2
  Dot Product/1 -> translational earth velocity (row 2)/1

== system chapter4_cascaded_nonlinear_closed_pid/Euler Transformation1/Transformation matrix T/Row3 of R ==
  translational body velocity : Inport
  angular position : Inport  Port=2
  -sY : Fcn  Expr=-sin(u[2])
  Dot Product : DotProduct  OutDataTypeStr=Inherit: Inherit via internal rule
  Mux1 : Mux  Inputs=3
  cY.cX : Fcn  Expr=cos(u[2])*cos(u[1])
  cY.sX : Fcn  Expr=cos(u[2])*sin(u[1])
  translational earth velocity (row 3) : Outport  InitialOutput=0
  wires:
  Mux1/1 -> Dot Product/1
  cY.cX/1 -> Mux1/3
  cY.sX/1 -> Mux1/2
  -sY/1 -> Mux1/1
  angular position/1 -> cY.cX/1, cY.sX/1, -sY/1
  translational body velocity/1 -> Dot Product/2
  Dot Product/1 -> translational earth velocity (row 3)/1

== system chapter4_cascaded_nonlinear_closed_pid/Euler Transformation1/Transformation matrix R/Row2 of T/Dot Product1 ==
